simulink model "SolarCar"  (R2025b)
settings: Solver=VariableStepAuto  StartTime=0.0  StopTime=10.0  RelTol=1e-3
undefined symbols (not defined in the file): Line
(part 2 of 2)

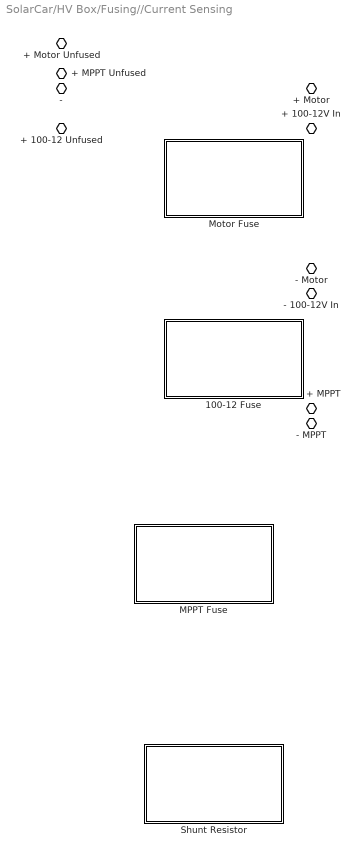
== system SolarCar/HV Box/Fusing//Current Sensing ==
  100-12 Fuse : Subsystem
      settings: PortSchema="{\"entries\":[{\"content\":{\"headerSize\":26,\"margin\":15,\"minimumSpacing\":25,\"sides\":[{\"content\":{},\"type\":\"ConnectorPlacement.EquallySpacedRectSide\",\"uuid\":\"16c5a28a-8204-43c6-ae1e-ca56bf00262c\"},{\"content\":{\"side\":\"RIGHT\"},\"type\":\"ConnectorPlacement.EquallySpacedRectSide\",\"uuid\":\"d50f7b79-0d90-4c13-9b04-ddd7ba1c0b17\"},{\"content\":{\"side\":\"TOP\"},\"type\":\"ConnectorPlacement.EquallySpacedRectSide\",\"uuid\":\"232c283e-7372-4332-942a-1b4711a4445f\"}]},\"type\":\"ConnectorPlacement.EquallySpacedConnector\",\"uuid\":\"38533706-c242-4f43-b565-c99062dd3fc1\"}],\"packageUris\":[\"http://schema.mathworks.com/mf0/Connector/R2020b\"],\"version\":\"1.0\"}"
  MPPT Fuse : Subsystem
      settings: PortSchema="{\"entries\":[{\"content\":{\"headerSize\":26,\"margin\":15,\"minimumSpacing\":25,\"sides\":[{\"content\":{},\"type\":\"ConnectorPlacement.EquallySpacedRectSide\",\"uuid\":\"16c5a28a-8204-43c6-ae1e-ca56bf00262c\"},{\"content\":{\"side\":\"RIGHT\"},\"type\":\"ConnectorPlacement.EquallySpacedRectSide\",\"uuid\":\"d50f7b79-0d90-4c13-9b04-ddd7ba1c0b17\"},{\"content\":{\"side\":\"TOP\"},\"type\":\"ConnectorPlacement.EquallySpacedRectSide\",\"uuid\":\"232c283e-7372-4332-942a-1b4711a4445f\"}]},\"type\":\"ConnectorPlacement.EquallySpacedConnector\",\"uuid\":\"38533706-c242-4f43-b565-c99062dd3fc1\"}],\"packageUris\":[\"http://schema.mathworks.com/mf0/Connector/R2020b\"],\"version\":\"1.0\"}"
  Motor Fuse : Subsystem
      settings: PortSchema="{\"entries\":[{\"content\":{\"headerSize\":26,\"margin\":15,\"minimumSpacing\":25,\"sides\":[{\"content\":{\"connectorIds\":[\"LConn1\"]},\"type\":\"ConnectorPlacement.EquallySpacedRectSide\",\"uuid\":\"16c5a28a-8204-43c6-ae1e-ca56bf00262c\"},{\"content\":{\"side\":\"RIGHT\"},\"type\":\"ConnectorPlacement.EquallySpacedRectSide\",\"uuid\":\"d50f7b79-0d90-4c13-9b04-ddd7ba1c0b17\"},{\"content\":{\"side\":\"TOP\"},\"type\":\"ConnectorPlacement.EquallySpacedRectSide\",\"uuid\":\"232c283e-7372-4332-942a-1b4711a4445f\"}]},\"type\":\"ConnectorPlacement.EquallySpacedConnector\",\"uuid\":\"38533706-c242-4f43-b565-c99062dd3fc1\"}],\"packageUris\":[\"http://schema.mathworks.com/mf0/Connector/R2020b\"],\"version\":\"1.0\"}"
  Shunt Resistor : Subsystem
      settings: PortSchema="{\"entries\":[{\"content\":{\"headerSize\":26,\"margin\":15,\"minimumSpacing\":25,\"sides\":[{\"content\":{},\"type\":\"ConnectorPlacement.EquallySpacedRectSide\",\"uuid\":\"16c5a28a-8204-43c6-ae1e-ca56bf00262c\"},{\"content\":{\"side\":\"RIGHT\"},\"type\":\"ConnectorPlacement.EquallySpacedRectSide\",\"uuid\":\"d50f7b79-0d90-4c13-9b04-ddd7ba1c0b17\"},{\"content\":{\"side\":\"TOP\"},\"type\":\"ConnectorPlacement.EquallySpacedRectSide\",\"uuid\":\"232c283e-7372-4332-942a-1b4711a4445f\"}]},\"type\":\"ConnectorPlacement.EquallySpacedConnector\",\"uuid\":\"38533706-c242-4f43-b565-c99062dd3fc1\"}],\"packageUris\":[\"http://schema.mathworks.com/mf0/Connector/R2020b\"],\"version\":\"1.0\"}"
  + Motor Unfused : PMIOPort  Side=Left
  + MPPT Unfused : PMIOPort  Port=2  Side=Left
  - : PMIOPort  Port=3  Side=Left
  + 100-12 Unfused : PMIOPort  Port=4  Side=Left
  + Motor : PMIOPort  Port=5  Side=Right
  + 100-12V In : PMIOPort  Port=6  Side=Right
  - Motor : PMIOPort  Port=7  Side=Right
  - 100-12V In : PMIOPort  Port=8  Side=Right
  + MPPT : PMIOPort  Port=9  Side=Right
  - MPPT : PMIOPort  Port=10  Side=Right

== system SolarCar/HV Box/Supercapacitor ==
  Bidirectional DC-DC : Subsystem
      settings: PortSchema="{\"entries\":[{\"content\":{\"headerSize\":26,\"margin\":15,\"minimumSpacing\":25,\"sides\":[{\"content\":{\"connectorIds\":[\"LConn1\",\"LConn2\"]},\"type\":\"ConnectorPlacement.EquallySpacedRectSide\",\"uuid\":\"7f164fa2-9272-4d7a-9d1b-73fbad559026\"},{\"content\":{\"connectorIds\":[\"RConn1\",\"RConn2\"],\"side\":\"RIGHT\"},\"type\":\"ConnectorPlacement.EquallySpacedRectSide\",\"uuid\":\"4e5c1bb6-197d-43aa-a880-a6796570230e\"},{\"content\":{\"side\":\"TOP\"},\"type\":\"ConnectorPlacement.EquallySpacedRectSide\",\"uuid\":\"a6abaace-1014-4cef-9d43-479b6863617c\"}]},\"type\":\"ConnectorPlacement.EquallySpacedConnector\",\"uuid\":\"97f01c5b-0fe0-4837-90bc-01d73eb3d078\"}],\"packageUris\":[\"http://schema.mathworks.com/mf0/Connector/R2020b\"],\"version\":\"1.0\"}"
  Supercapacitor : Subsystem
      settings: PortSchema="{\"entries\":[{\"content\":{\"headerSize\":26,\"margin\":15,\"minimumSpacing\":25,\"sides\":[{\"content\":{\"connectorIds\":[\"LConn1\",\"LConn2\"]},\"type\":\"ConnectorPlacement.EquallySpacedRectSide\",\"uuid\":\"7f164fa2-9272-4d7a-9d1b-73fbad559026\"},{\"content\":{\"side\":\"RIGHT\"},\"type\":\"ConnectorPlacement.EquallySpacedRectSide\",\"uuid\":\"4e5c1bb6-197d-43aa-a880-a6796570230e\"},{\"content\":{\"side\":\"TOP\"},\"type\":\"ConnectorPlacement.EquallySpacedRectSide\",\"uuid\":\"a6abaace-1014-4cef-9d43-479b6863617c\"}]},\"type\":\"ConnectorPlacement.EquallySpacedConnector\",\"uuid\":\"97f01c5b-0fe0-4837-90bc-01d73eb3d078\"}],\"packageUris\":[\"http://schema.mathworks.com/mf0/Connector/R2020b\"],\"version\":\"1.0\"}"
  + Motor : PMIOPort  Side=Left
  - Motor : PMIOPort  Port=2  Side=Left
  connections:
  Bidirectional DC-DC/RConn1 -- Supercapacitor/LConn1
  Bidirectional DC-DC/RConn2 -- Supercapacitor/LConn2
  + Motor/RConn1 -- Bidirectional DC-DC/LConn1
  - Motor/RConn1 -- Bidirectional DC-DC/LConn2

== system SolarCar/LV Box/12-5V ==
  12V Fuse Board Out : PMIOPort  Side=Left
  GND Fuse Board Out : PMIOPort  Port=2  Side=Left
  5V 12-5 Out : PMIOPort  Port=3  Side=Right

== system SolarCar/LV Box/Battery Charger ==
  + Supplemental : PMIOPort  Side=Left
  - Supplemental : PMIOPort  Port=2  Side=Left
  + 100-12V Out : PMIOPort  Port=3  Side=Right
  - 100-12V Out : PMIOPort  Port=4  Side=Right

== system SolarCar/LV Box/CAN Hub ==
  Essentials CANH : PMIOPort  Side=Left
  Essentials CANL : PMIOPort  Port=2  Side=Left
  Telemetry CANH : PMIOPort  Port=3  Side=Left
  Telemetry CANL : PMIOPort  Port=4  Side=Left
  5V Fuse Board Out : PMIOPort  Port=5  Side=Left
  GND Fuse Board Out : PMIOPort  Port=6  Side=Left

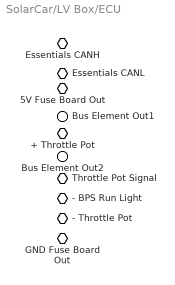
== system SolarCar/LV Box/ECU ==
  Essentials CANH : PMIOPort  Side=Left
  Essentials CANL : PMIOPort  Port=2  Side=Left
  5V Fuse Board Out : PMIOPort  Port=3  Side=Left
  GND Fuse Board Out : PMIOPort  Port=4  Side=Left
  + Throttle Pot : PMIOPort  Port=5  Side=Left
  Throttle Pot Signal : PMIOPort  Port=6  Side=Left
  - Throttle Pot : PMIOPort  Port=7  Side=Left
  - BPS Run Light : PMIOPort  Port=8  Side=Right
  Bus Element Out1 : Outport  PortName=Throttle Signal
  Bus Element Out2 : Outport  Port=2  PortName=Regen Signal

== system SolarCar/LV Box/Fuse Board ==
  + MUX Out : PMIOPort  Side=Left
  - MUX Out : PMIOPort  Port=2  Side=Left
  12V Fuse Board Out : PMIOPort  Port=3  Side=Right
  5V Fuse Board Out : PMIOPort  Port=4  Side=Right
  GND Fuse Board Out : PMIOPort  Port=5  Side=Right
  5V 12-5 Out : PMIOPort  Port=6  Side=Left

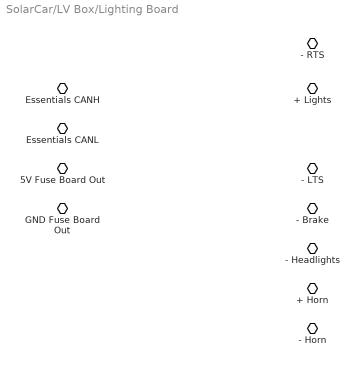
== system SolarCar/LV Box/Lighting Board ==
  Essentials CANH : PMIOPort  Side=Left
  Essentials CANL : PMIOPort  Port=2  Side=Left
  - RTS : PMIOPort  Port=3  Side=Right
  + Lights : PMIOPort  Port=4  Side=Right
  - LTS : PMIOPort  Port=5  Side=Right
  - Brake : PMIOPort  Port=6  Side=Right
  - Headlights : PMIOPort  Port=7  Side=Right
  + Horn : PMIOPort  Port=8  Side=Right
  - Horn : PMIOPort  Port=9  Side=Right
  5V Fuse Board Out : PMIOPort  Port=10  Side=Left
  GND Fuse Board Out : PMIOPort  Port=11  Side=Left

== system SolarCar/LV Box/Power MUX ==
  + 12V Supplemental : PMIOPort  Side=Left
  GND Supplemental : PMIOPort  Port=2  Side=Left
  + 100-12V Out : PMIOPort  Port=3  Side=Left
  + MUX Out : PMIOPort  Port=4  Side=Right
  - MUX Out : PMIOPort  Port=5  Side=Right
  - 100-12V Out : PMIOPort  Port=6  Side=Right

== system SolarCar/LV Box/Supplemental Battery ==
  + Supplemental : PMIOPort  Side=Right
  - Supplemental : PMIOPort  Port=2  Side=Right

== system SolarCar/Motor//Controller/Motor ==
  A : PMIOPort  Side=Left
  B : PMIOPort  Port=2  Side=Left
  C : PMIOPort  Port=3  Side=Left
  Data : PMIOPort  Port=4  Side=Left

== system SolarCar/Motor//Controller/Motor Controller ==
  Bus Element In1 : Inport  PortName=Terminal
  + Motor : PMIOPort  Side=Left
  - Motor : PMIOPort  Port=2  Side=Left
  A : PMIOPort  Port=3  Side=Right
  B : PMIOPort  Port=4  Side=Right
  C : PMIOPort  Port=5  Side=Right
  Data : PMIOPort  Port=6  Side=Right

== system SolarCar/Motor//Controller/Terminal ==
  Bus Element In1 : Inport  PortName=Regen Signal
  Bus Element In2 : Inport  Port=2  PortName=Throttle Signal
  Forward/Reverse Out : PMIOPort  Side=Left
  Forward/Reverse In : PMIOPort  Port=2  Side=Left
  Bus Element Out1 : Outport  PortName=Terminal

== system SolarCar/Top Shell/Array ==
  Vpv+ : PMIOPort  Side=Right
  Vpv- : PMIOPort  Port=2  Side=Right

== system SolarCar/Top Shell/MPPT x4 ==
  + MPPT : PMIOPort  Side=Right
  - MPPT : PMIOPort  Port=2  Side=Right
  12V : PMIOPort  Port=3  Side=Right
  GND : PMIOPort  Port=4  Side=Right
  Essentials CANH : PMIOPort  Port=5  Side=Right
  Essentials CANL : PMIOPort  Port=6  Side=Right
  Vpv+ : PMIOPort  Port=7  Side=Left
  Vpv- : PMIOPort  Port=8  Side=Left

== system SolarCar/Dispersed/Lights/BPS Run Light ==
  + Lights : PMIOPort  Side=Left
  - BPS Run Light : PMIOPort  Port=2  Side=Left

== system SolarCar/Dispersed/Lights/Brake Lights ==
  + Lights : PMIOPort  Side=Left
  - Brake : PMIOPort  Port=2  Side=Left

== system SolarCar/Dispersed/Lights/Headlights ==
  + Lights : PMIOPort  Side=Left
  - Headlights : PMIOPort  Port=2  Side=Left

== system SolarCar/Dispersed/Lights/Left Turn Signal ==
  + Lights : PMIOPort  Side=Left
  - LTS : PMIOPort  Port=2  Side=Left

== system SolarCar/Dispersed/Lights/Right Turn Signal ==
  Bus Element In1 : Inport  PortName=InBus
  + Lights : PMIOPort  Side=Left

== system SolarCar/HV Box/Contactors/+ MPPT Contactor ==
  Bus Element In2 : Inport  PortName=+ MPPT Coil
  Bus Element In3 : Inport  Port=2  PortName=- MPPT Coil
  Bus Element In1 : Inport  Port=3  PortName=+ Line
  + MPPT : PMIOPort  Side=Right

== system SolarCar/HV Box/Contactors/+ Motor Contactor ==
  Bus Element In2 : Inport  PortName=InBus
  Bus Element In3 : Inport  Port=2  PortName=- Motor Coil
  Bus Element In1 : Inport  Port=3  PortName=+ Line
  + Motor : PMIOPort  Side=Right

== system SolarCar/HV Box/Contactors/+ Precharge MPPT Contactor ==
  Bus Element In2 : Inport  PortName=+ Precharge MPPT Coil
  Bus Element In3 : Inport  Port=2  PortName=- Precharge MPPT Coil
  Bus Element In1 : Inport  Port=3  PortName=+ Line
  + MPPT : PMIOPort  Side=Right

== system SolarCar/HV Box/Contactors/+ Precharge Motor Contactor ==
  Bus Element In2 : Inport  PortName=+ Precharge Motor Coil
  Bus Element In3 : Inport  Port=2  PortName=InBus
  Bus Element In1 : Inport  Port=3  PortName=+ Line
  + Motor : PMIOPort  Side=Right

== system SolarCar/HV Box/Contactors/- Main Contactor ==
  Bus Element In3 : Inport  PortName=+ Main Coil
  Bus Element In4 : Inport  Port=2  PortName=- Main Coil
  Bus Element In2 : Inport  Port=3  PortName=+ Line
  Bus Element In1 : Inport  Port=4  PortName=- Line
  - : PMIOPort  Side=Right

== system SolarCar/HV Box/Fusing//Current Sensing/100-12 Fuse ==

== system SolarCar/HV Box/Fusing//Current Sensing/MPPT Fuse ==

== system SolarCar/HV Box/Fusing//Current Sensing/Motor Fuse ==
  + Motor : PMIOPort  Side=Left

== system SolarCar/HV Box/Fusing//Current Sensing/Shunt Resistor ==

== system SolarCar/HV Box/Supercapacitor/Bidirectional DC-DC ==
  + Supercapacitor : PMIOPort  Side=Right
  - Supercapacitor : PMIOPort  Port=2  Side=Right
  + Motor : PMIOPort  Port=3  Side=Left
  - Motor : PMIOPort  Port=4  Side=Left

== system SolarCar/HV Box/Supercapacitor/Supercapacitor ==
  + Supercapacitor : PMIOPort  Side=Left
  - Supercapacitor : PMIOPort  Port=2  Side=Left
